simulink model "diag_monitor"  (R2022b)
settings: Solver=FixedStepDiscrete  StartTime=0.0  StopTime=6  FixedStep=D.Ts  RelTol=1e-3
undefined symbols (not defined in the file or in its folder): D
settings Model: Creator=Mohamed Mehdi Hamdi  LastModifiedBy=Mohamed Mehdi Hamdi

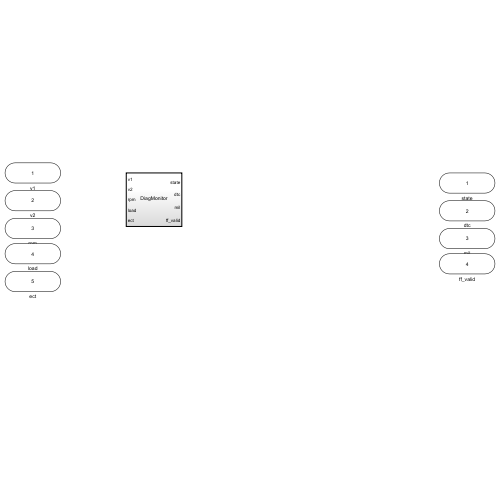
[thumbnail: Simulink's stored preview of the top-level diagram]
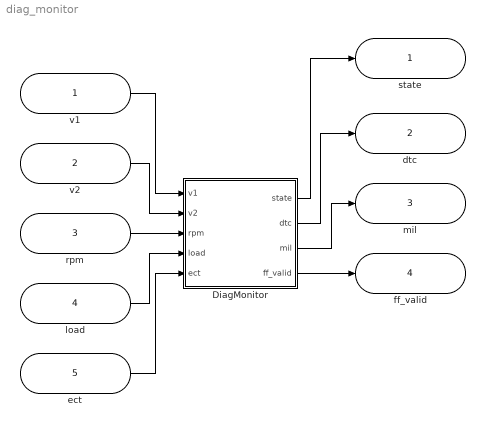
== system diag_monitor ==
  v1 : Inport
  v2 : Inport  Port=2
  rpm : Inport  Port=3
  load : Inport  Port=4
  ect : Inport  Port=5
  DiagMonitor : Subsystem  TreatAsAtomicUnit=on
  state : Outport
  dtc : Outport  Port=2
  mil : Outport  Port=3
  ff_valid : Outport  Port=4
  wires:
  v1/1 -> DiagMonitor/1(v1)
  rpm/1 -> DiagMonitor/3(rpm)
  v2/1 -> DiagMonitor/2(v2)
  ect/1 -> DiagMonitor/5(ect)
  load/1 -> DiagMonitor/4(load)
  DiagMonitor/2(dtc) -> dtc/1
  DiagMonitor/1(state) -> state/1
  DiagMonitor/3(mil) -> mil/1
  DiagMonitor/4(ff_valid) -> ff_valid/1

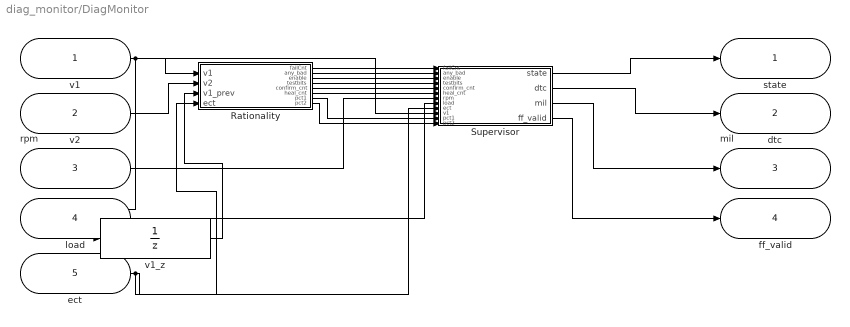
== system diag_monitor/DiagMonitor ==
  v1 : Inport
  v2 : Inport  Port=2
  rpm : Inport  Port=3
  load : Inport  Port=4
  ect : Inport  Port=5
  Rationality : MATLAB Function  TreatAsAtomicUnit=on
  Supervisor : Stateflow chart  TreatAsAtomicUnit=on
  v1_z : UnitDelay  SampleTime=D.Ts  HasFrameUpgradeWarning=on
  state : Outport
  dtc : Outport  Port=2
  mil : Outport  Port=3
  ff_valid : Outport  Port=4
  wires:
  v1/1 -> Rationality/1(v1), v1_z/1, Supervisor/10(v1)
  v2/1 -> Rationality/2(v2)
  v1_z/1 -> Rationality/3(v1_prev)
  ect/1 -> Rationality/4(ect), Supervisor/9(ect)
  rpm/1 -> Supervisor/7(rpm)
  load/1 -> Supervisor/8(load)
  Rationality/1(failCnt) -> Supervisor/1(failCnt)
  Rationality/2(any_bad) -> Supervisor/2(any_bad)
  Rationality/3(enable) -> Supervisor/3(enable)
  Rationality/4(testbits) -> Supervisor/4(testbits)
  Rationality/5(confirm_cnt) -> Supervisor/5(confirm_cnt)
  Rationality/6(heal_cnt) -> Supervisor/6(heal_cnt)
  Rationality/7(pct1) -> Supervisor/11(pct1)
  Rationality/8(pct2) -> Supervisor/12(pct2)
  Supervisor/1(state) -> state/1
  Supervisor/2(dtc) -> dtc/1
  Supervisor/3(mil) -> mil/1
  Supervisor/4(ff_valid) -> ff_valid/1

== matlab function diag_monitor/DiagMonitor/Rationality ==
  data: v1 input; failCnt output; v2 input; v1_prev input; ect input; any_bad output; enable output; testbits output; confirm_cnt output; heal_cnt output; pct1 output; pct2 output
function [failCnt, any_bad, enable, testbits, confirm_cnt, heal_cnt, pct1, pct2] = Rationality(v1, v2, v1_prev, ect)
%#codegen
%  Range + rate + correlation rationality tests with a shared debounced
%  fail counter. Counter is frozen unless enable conditions are met. Also
%  forwards the confirm/heal thresholds and the normalised percentages so
%  the supervisor can latch the DTC and capture the freeze-frame.
D = diag_const();
persistent fc prev_valid;
if isempty(fc); fc = 0; end
if isempty(prev_valid); prev_valid = false; end

pct1 = (v1 - D.v1_lo) / (D.v1_hi - D.v1_lo) * 100;
pct2 = (v2 - D.v2_lo) / (D.v2_hi - D.v2_lo) * 100;

range_bad = (v1 < D.v_oor_lo) || (v1 > D.v_oor_hi);
rate_bad  = prev_valid && (abs(v1 - v1_prev) > D.dv_max);
prev_valid = true;
corr_bad  = abs(pct1 - pct2) > D.corr_tol;
any_bad   = range_bad || rate_bad || corr_bad;
testbits  = uint8(range_bad) + uint8(2)*uint8(rate_bad) + uint8(4)*uint8(corr_bad);

enable = ect >= D.warm_min;
if enable
    if any_bad; fc = min(fc + 1, D.confirm_cnt); else; fc = max(fc - 1, 0); end
end
failCnt     = fc;
confirm_cnt = D.confirm_cnt;
heal_cnt    = D.heal_cnt;
end

== stateflow chart diag_monitor/DiagMonitor/Supervisor ==
  settings: updateMethod=DISCRETE  sampleTime=D.Ts
  state NO_FAULT
    en: state = uint8(0); mil = false;
    dtc = uint8(0); ff_valid = false; healCnt = 0;
  state PENDING
    en: state = uint8(1); mil = false;
  state CONFIRMED
    en: state = uint8(2); mil = true;
    if ~ff_valid
    dtc = testbits;
    ff_rpm = rpm; ff_load = load; ff_ect = ect;
    ff_v1 = v1; ff_pct1 = pct1; ff_pct2 = pct2;
    ff_valid = true;
    end
    du: dtc = bitor(dtc, testbits);
  state HEALING
    en: state = uint8(3); mil = true; healCnt = 0;
    du: healCnt = healCnt + 1;
  (default) -> NO_FAULT
  HEALING -> NO_FAULT [order 2] : [healCnt >= heal_cnt]
  PENDING -> NO_FAULT [order 2] : [failCnt == 0]
  NO_FAULT -> PENDING : [failCnt > 0]
  PENDING -> CONFIRMED [order 1] : [failCnt >= confirm_cnt]
  HEALING -> CONFIRMED [order 1] : [any_bad]
  CONFIRMED -> HEALING : [enable && ~any_bad]
  data: failCnt input double; any_bad input boolean; enable input boolean; testbits input uint8; confirm_cnt input double; heal_cnt input double; rpm input double; load input double; ect input double; v1 input double; pct1 input double; pct2 input double; state output uint8; dtc output uint8; mil output boolean; ff_valid output boolean; healCnt local double; ff_rpm local double; ff_load local double; ff_ect local double; ff_v1 local double; ff_pct1 local double; ff_pct2 local double
